simulink model "W12_PolePlacement"  (R2024b)
settings: Solver=ode45  StartTime=0.0  StopTime=t_end  MaxStep=0.005  RelTol=1e-3
PreLoadFcn:
  | % W12_PolePlacement 기본 파라미터 (모델을 열 때 자동 실행)
  | % 기본 예제 : DC 모터 위치제어 + 극배치 [-8 -10 -12]
  | %
  | % [주의] setup_path 를 안 한 상태에서 모델만 열어도 돌아가야 합니다.
  | %        경로가 없으면 plant_dcmotor 를 못 찾으므로 아래처럼 숫자로 대신합니다.
  | %        (숫자는 plant_dcmotor(''position'') 이 주는 값과 같습니다)
  | if isempty(which('plant_dcmotor'))
  |     pp = struct('A', [0 1 0; 0 -10 1; 0 -0.02 -2], ...
  |                 'B', [0; 0; 2], 'C', [1 0 0], 'D', 0);
  | else
  |     [~, pp] = plant_dcmotor('position');
  | end
  | A_mat = pp.A;  B_mat = pp.B;
  | K_fb  = place(pp.A, pp.B, [-8 -10 -12]);
  | Kr    = 1/dcgain(ss(pp.A - pp.B*K_fb, pp.B, pp.C, pp.D));
  | x0    = zeros(size(A_mat,1),1);
  | r_amp = 1;  u_lim = 1e6;  t_end = 1.5;
  | clear pp
settings Model: Creator=admin  LastModifiedBy=admin

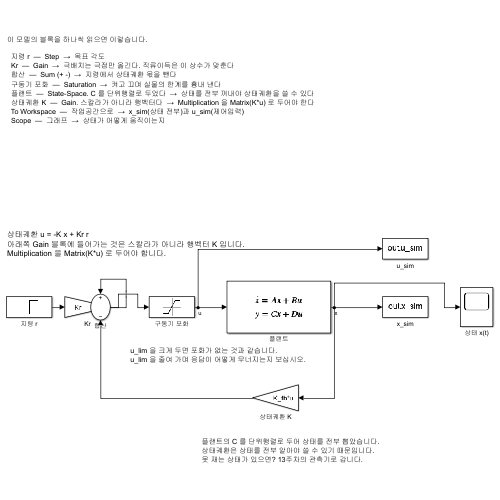
[thumbnail: Simulink's stored preview of the top-level diagram]
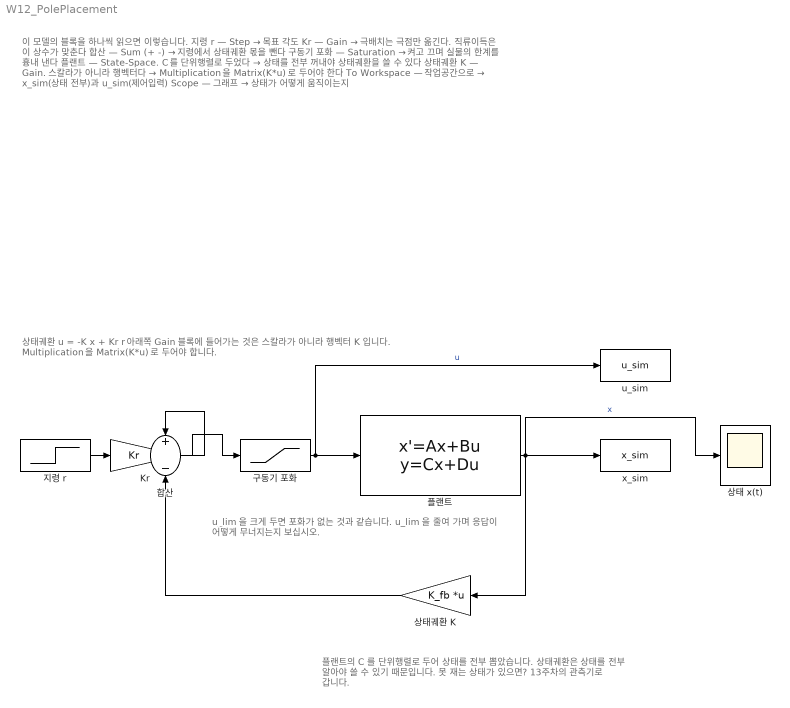
== system W12_PolePlacement ==
  note: 상태궤환 u = -K x + Kr r
      | 아래쪽 Gain 블록에 들어가는 것은 스칼라가 아니라 행벡터 K 입니다.
      | Multiplication 을 Matrix(K*u) 로 두어야 합니다.
  note: 플랜트의 C 를 단위행렬로 두어 상태를 전부 뽑았습니다.
      | 상태궤환은 상태를 전부 알아야 쓸 수 있기 때문입니다.
      | 못 재는 상태가 있으면? 13주차의 관측기로 갑니다.
  note: u_lim 을 크게 두면 포화가 없는 것과 같습니다.
      | u_lim 을 줄여 가며 응답이 어떻게 무너지는지 보십시오.
  note: 이 모델의 블록을 하나씩 읽으면 이렇습니다.
      |
      |   지령 r  —  Step  →  목표 각도
      |   Kr  —  Gain  →  극배치는 극점만 옮긴다. 직류이득은 이 상수가 맞춘다
      |   합산  —  Sum (+ -)  →  지령에서 상태궤환 몫을 뺀다
      |   구동기 포화  —  Saturation  →  켜고 끄며 실물의 한계를 흉내 낸다
      |   플랜트  —  State-Space. C 를 단위행렬로 두었다  →  상태를 전부 꺼내야 상태궤환을 쓸 수 있다
      |   상태궤환 K  —  Gain. 스칼라가 아니라 행벡터다  →  Multiplication 을 Matrix(K*u) 로 두어야 한다
      |   To Workspace  —  작업공간으로  →  x_sim(상태 전부)과 u_sim(제어입력)
      |   Scope  —  그래프  →  상태가 어떻게 움직이는지
  Kr : Gain  Gain=Kr
  u_sim : ToWorkspace  VariableName=u_sim  SaveFormat=Timeseries  SampleTime=-1
  x_sim : ToWorkspace  VariableName=x_sim  SaveFormat=Timeseries  SampleTime=-1
  구동기 포화 : Saturate  UpperLimit=u_lim  LowerLimit=-u_lim
  상태 x(t) : Scope
  상태궤환 K : Gain  Gain=K_fb  Multiplication=Matrix(K*u)
  지령 r : Step  Time=0  After=r_amp  SampleTime=0
  플랜트 : StateSpace  A=A_mat  B=B_mat  C=eye(size(A_mat,1))  D=zeros(size(A_mat,1),1)  InitialCondition=x0
  합산 : Sum  Inputs=+-
  wires:
  지령 r/1 -> Kr/1
  Kr/1 -> 합산/1
  합산/1 -> 구동기 포화/1
  구동기 포화/1 -> 플랜트/1, u_sim/1  "u"
  플랜트/1 -> x_sim/1, 상태 x(t)/1, 상태궤환 K/1  "x"
  상태궤환 K/1 -> 합산/2
